simulink subsystem "PowerSplitGeartrain_refsub_Basic"  (R2023a)
settings: Solver=VariableStepAuto  StartTime=0.0  StopTime=10.0  RelTol=1e-3
libraries: sdl_lib x4
settings Model: Creator=isaacito  LastModifiedBy=isaacito
settings SolverCC: AlgebraicLoopSolver=TrustRegion
settings OptimizationCC: ReuseModelBlockBuffer=off
settings DebuggingCC: UnconnectedInputMsg=warning  UnconnectedOutputMsg=warning  UnconnectedLineMsg=warning
settings ModelReferenceCC: EnableRefExpFcnMdlSchedulingChecks=on
settings RTWCC: DLArmComputeVersion=19.05

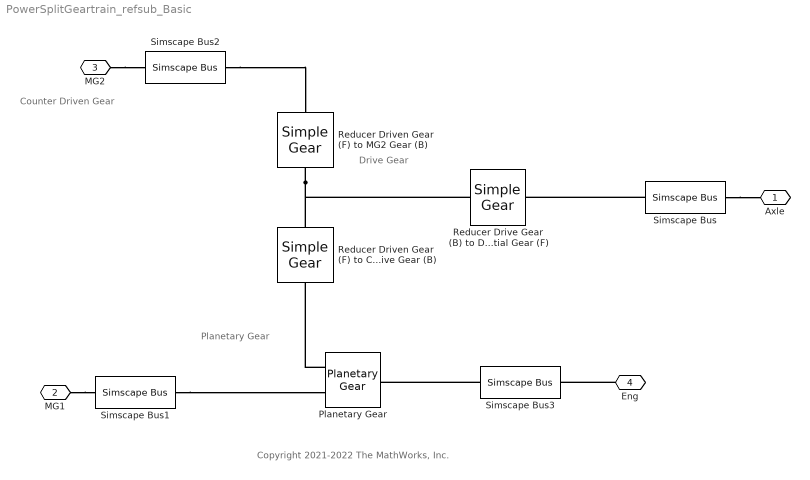
== system PowerSplitGeartrain_refsub_Basic ==
  note: Copyright 2021-2022 The MathWorks, Inc.
  note: Counter Driven Gear
  note: Drive Gear
  note: Planetary Gear
  Planetary Gear : sdl_lib/Gears/Planetary Gear  rs_ratio=powerSplit.planetary_ringToSunGearRatio  friction_model=sdl.enum.gear_friction.constant  efficiency=powerSplit.planetary_efficiencies  temperature_TLU=[280, 300, 320] K  efficiency_sp_TLU=[.95, .9, .85]  efficiency_rp_TLU=[.95, .9, .85]  pwr_thr=smoothing.planetary_meshing_loss_thresholds_W W  mu_visc=powerSplit.planetary_frictions_Nm_per_rpm m*N/rpm  model_inertia=simscape.enum.onoff.on  planet_inertia=powerSplit.planetary_planetGearInertia_kg_m2 kg*m^2  thermal_mass=50 J/K  T_init=300 K
  Reducer Drive Gear (B) to Differential Gear (F) : sdl_lib/Gears/Simple Gear  ratio=powerSplit.reducer_differentialGearRatio  rotation_direction=sdl.enum.shaftOutputDirection.opposite  friction_model=sdl.enum.gear_efficiencies_load.constant  T_noload=0.1 N*m  T_nom=5 N*m  efficiency_nom=0.8  efficiency=powerSplit.reducer_efficiency  temperature_TLU=[280, 300, 320] K  load_TLU=[1, 5, 10] N*m  efficiency_TLU=[.95, .9, .85]  efficiency_TLU2=[.85, .8, .75; .95, .9, .85; .85, .8, .7]  w_thr=0.01 rad/s  pwr_thr=smoothing.gear_meshing_loss_threshold_W W  backlash_model=sdl.enum.backlashModel.Off  backlash_distance=1e-3 mm  x0=0 mm  r_base=0.1 m  hardstop_model=simscape.enum.hardstop.smooth  transition=1e-4 mm  backlash_stiffness=1e7 N/m  backlash_damping=1e6 N*s/m  e=0  v_tol=0.001 m/s  mu_visc=powerSplit.reducer_friction_Nm_per_rpm N*m/(rad/s)  enable_faults=simscape.enum.onoff.off  efficiency_fault=0.05  external_fault=simscape.enum.onoff.off  temporal_fault=simscape.enum.onoff.off  fault_time=5 s  fault_angles=pi / 12 rad  report_fault=simscape.enum.assert.action.none  thermal_mass=50 J/K  temperature_specify=off  temperature_priority=High  temperature=300 K  temperature_nominal_specify=off  temperature_nominal_unit=K  temperature_nominal_value=1  x_backlash_specify=off  x_backlash_priority=None  x_backlash=0 mm  x_backlash_nominal_specify=off  x_backlash_nominal_unit=mm  x_backlash_nominal_value=1  f_hardstop_specify=off  f_hardstop_priority=None  f_hardstop=0 N  f_hardstop_nominal_specify=off  f_hardstop_nominal_unit=N  f_hardstop_nominal_value=1  v_backlash_specify=off  v_backlash_priority=None  v_backlash=0 m/s  v_backlash_nominal_specify=off  v_backlash_nominal_unit=m/s  v_backlash_nominal_value=1
  Reducer Driven Gear (F) to Counter Drive Gear (B) : sdl_lib/Gears/Simple Gear  ratio=powerSplit.reducer_counterDriveGearRatio  rotation_direction=sdl.enum.shaftOutputDirection.opposite  friction_model=sdl.enum.gear_efficiencies_load.constant  T_noload=0.1 N*m  T_nom=5 N*m  efficiency_nom=0.8  efficiency=powerSplit.reducer_efficiency  temperature_TLU=[280, 300, 320] K  load_TLU=[1, 5, 10] N*m  efficiency_TLU=[.95, .9, .85]  efficiency_TLU2=[.85, .8, .75; .95, .9, .85; .85, .8, .7]  w_thr=0.01 rad/s  pwr_thr=smoothing.gear_meshing_loss_threshold_W W  backlash_model=sdl.enum.backlashModel.Off  backlash_distance=1e-3 mm  x0=0 mm  r_base=0.1 m  hardstop_model=simscape.enum.hardstop.smooth  transition=1e-4 mm  backlash_stiffness=1e7 N/m  backlash_damping=1e6 N*s/m  e=0  v_tol=0.001 m/s  mu_visc=powerSplit.reducer_friction_Nm_per_rpm N*m/(rad/s)  enable_faults=simscape.enum.onoff.off  efficiency_fault=0.05  external_fault=simscape.enum.onoff.off  temporal_fault=simscape.enum.onoff.off  fault_time=5 s  fault_angles=pi / 12 rad  report_fault=simscape.enum.assert.action.none  thermal_mass=50 J/K  temperature_specify=off  temperature_priority=High  temperature=300 K  temperature_nominal_specify=off  temperature_nominal_unit=K  temperature_nominal_value=1  x_backlash_specify=off  x_backlash_priority=None  x_backlash=0 mm  x_backlash_nominal_specify=off  x_backlash_nominal_unit=mm  x_backlash_nominal_value=1  f_hardstop_specify=off  f_hardstop_priority=None  f_hardstop=0 N  f_hardstop_nominal_specify=off  f_hardstop_nominal_unit=N  f_hardstop_nominal_value=1  v_backlash_specify=off  v_backlash_priority=None  v_backlash=0 m/s  v_backlash_nominal_specify=off  v_backlash_nominal_unit=m/s  v_backlash_nominal_value=1
  Reducer Driven Gear (F) to MG2 Gear (B) : sdl_lib/Gears/Simple Gear  ratio=powerSplit.reducer_MG2GearRatio  rotation_direction=sdl.enum.shaftOutputDirection.opposite  friction_model=sdl.enum.gear_efficiencies_load.constant  T_noload=0.1 N*m  T_nom=5 N*m  efficiency_nom=0.8  efficiency=powerSplit.reducer_efficiency  temperature_TLU=[280, 300, 320] K  load_TLU=[1, 5, 10] N*m  efficiency_TLU=[.95, .9, .85]  efficiency_TLU2=[.85, .8, .75; .95, .9, .85; .85, .8, .7]  w_thr=0.01 rad/s  pwr_thr=smoothing.gear_meshing_loss_threshold_W W  backlash_model=sdl.enum.backlashModel.Off  backlash_distance=1e-3 mm  x0=0 mm  r_base=0.1 m  hardstop_model=simscape.enum.hardstop.smooth  transition=1e-4 mm  backlash_stiffness=1e7 N/m  backlash_damping=1e6 N*s/m  e=0  v_tol=0.001 m/s  mu_visc=powerSplit.reducer_friction_Nm_per_rpm m*N/rpm  enable_faults=simscape.enum.onoff.off  efficiency_fault=0.05  external_fault=simscape.enum.onoff.off  temporal_fault=simscape.enum.onoff.off  fault_time=5 s  fault_angles=pi / 12 rad  report_fault=simscape.enum.assert.action.none  thermal_mass=50 J/K  temperature_specify=off  temperature_priority=High  temperature=300 K  temperature_nominal_specify=off  temperature_nominal_unit=K  temperature_nominal_value=1  x_backlash_specify=off  x_backlash_priority=None  x_backlash=0 mm  x_backlash_nominal_specify=off  x_backlash_nominal_unit=mm  x_backlash_nominal_value=1  f_hardstop_specify=off  f_hardstop_priority=None  f_hardstop=0 N  f_hardstop_nominal_specify=off  f_hardstop_nominal_unit=N  f_hardstop_nominal_value=1  v_backlash_specify=off  v_backlash_priority=None  v_backlash=0 m/s  v_backlash_nominal_specify=off  v_backlash_nominal_unit=m/s  v_backlash_nominal_value=1
  Simscape Bus{,1..3} (4 alike) : SimscapeBus  HierarchyStrings=AngSpd  ConnectionType=Bus: Bus_Rotational
      settings: AttributesFormatString=%<ConnectionType>
  Axle : PMIOPort  Side=Left
  MG1 : PMIOPort  Port=2  Side=Left
  MG2 : PMIOPort  Port=3  Side=Left
  Eng : PMIOPort  Port=4  Side=Left
  connections:
  Reducer Driven Gear (F) to MG2 Gear (B)/RConn1 -- Reducer Drive Gear (B) to Differential Gear (F)/RConn1 -- Reducer Driven Gear (F) to Counter Drive Gear (B)/RConn1
  Planetary Gear/RConn1 -- Reducer Driven Gear (F) to Counter Drive Gear (B)/LConn1
  Simscape Bus/LConn1 -- Reducer Drive Gear (B) to Differential Gear (F)/LConn1
  Simscape Bus2/LConn1 -- Reducer Driven Gear (F) to MG2 Gear (B)/LConn1
  Simscape Bus1/LConn1 -- Planetary Gear/RConn2
  Simscape Bus3/LConn1 -- Planetary Gear/LConn1
  Simscape Bus/RConn1 -- Axle/RConn1
  MG1/RConn1 -- Simscape Bus1/RConn1
  MG2/RConn1 -- Simscape Bus2/RConn1
  Eng/RConn1 -- Simscape Bus3/RConn1
